simulink model "rfdc"  (R2021a)
settings: Solver=VariableStepAuto  StartTime=0.0  StopTime=10.0  RelTol=1e-3
libraries: xbsIndex_r4 x8
(part 3 of 3)

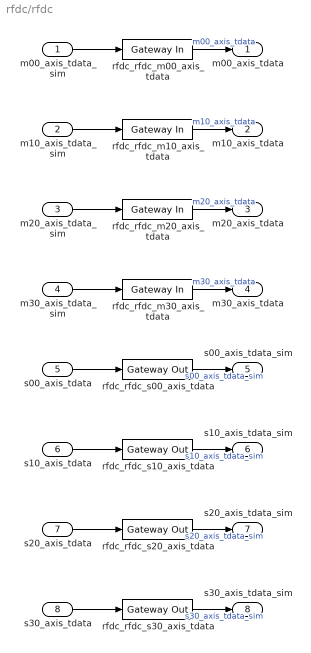
== system rfdc/rfdc ==
  m00_axis_tdata_sim : Inport
  m10_axis_tdata_sim : Inport  Port=2
  m20_axis_tdata_sim : Inport  Port=3
  m30_axis_tdata_sim : Inport  Port=4
  s00_axis_tdata : Inport  Port=5
  s10_axis_tdata : Inport  Port=6
  s20_axis_tdata : Inport  Port=7
  s30_axis_tdata : Inport  Port=8
  rfdc_rfdc_m00_axis_tdata : xbsIndex_r4/Gateway In  gui_display_data_type=Fixed-point  arith_type="Signed  (2's comp)"  n_bits=128  bin_pt=0  preci_type=Single  exp_width=8  frac_width=24  rows=1  columns=1  quantization="Round  (unbiased: +/- Inf)"  overflow=Saturate  period=1  UseAsADC=off  ADCChannel='1'  interface=None  automatic_assignment=on  address_offset=hex2dec('00')  intf_name=''  intf_description=''  default_value=0  timing_constraint=None  locs_specified=off  LOCs={}  io_standard={}  inherit_from_input=off  hdl_port=on  dbl_ovrd=off  block_type=gatewayin
  rfdc_rfdc_m10_axis_tdata : xbsIndex_r4/Gateway In  gui_display_data_type=Fixed-point  arith_type="Signed  (2's comp)"  n_bits=128  bin_pt=0  preci_type=Single  exp_width=8  frac_width=24  rows=1  columns=1  quantization="Round  (unbiased: +/- Inf)"  overflow=Saturate  period=1  UseAsADC=off  ADCChannel='1'  interface=None  automatic_assignment=on  address_offset=hex2dec('00')  intf_name=''  intf_description=''  default_value=0  timing_constraint=None  locs_specified=off  LOCs={}  io_standard={}  inherit_from_input=off  hdl_port=on  dbl_ovrd=off  block_type=gatewayin
  rfdc_rfdc_m20_axis_tdata : xbsIndex_r4/Gateway In  gui_display_data_type=Fixed-point  arith_type="Signed  (2's comp)"  n_bits=128  bin_pt=0  preci_type=Single  exp_width=8  frac_width=24  rows=1  columns=1  quantization="Round  (unbiased: +/- Inf)"  overflow=Saturate  period=1  UseAsADC=off  ADCChannel='1'  interface=None  automatic_assignment=on  address_offset=hex2dec('00')  intf_name=''  intf_description=''  default_value=0  timing_constraint=None  locs_specified=off  LOCs={}  io_standard={}  inherit_from_input=off  hdl_port=on  dbl_ovrd=off  block_type=gatewayin
  rfdc_rfdc_m30_axis_tdata : xbsIndex_r4/Gateway In  gui_display_data_type=Fixed-point  arith_type="Signed  (2's comp)"  n_bits=128  bin_pt=0  preci_type=Single  exp_width=8  frac_width=24  rows=1  columns=1  quantization="Round  (unbiased: +/- Inf)"  overflow=Saturate  period=1  UseAsADC=off  ADCChannel='1'  interface=None  automatic_assignment=on  address_offset=hex2dec('00')  intf_name=''  intf_description=''  default_value=0  timing_constraint=None  locs_specified=off  LOCs={}  io_standard={}  inherit_from_input=off  hdl_port=on  dbl_ovrd=off  block_type=gatewayin
  rfdc_rfdc_s00_axis_tdata : xbsIndex_r4/Gateway Out  inherit_from_input=off  hdl_port=on  rows=1  columns=1  UseAsDAC=off  DACChannel='1'  interface=None  automatic_assignment=on  address_offset=hex2dec('00')  intf_name=''  intf_description=''  timing_constraint=None  locs_specified=off  LOCs={}  io_standard={}  block_type=gatewayout
  rfdc_rfdc_s10_axis_tdata : xbsIndex_r4/Gateway Out  inherit_from_input=off  hdl_port=on  rows=1  columns=1  UseAsDAC=off  DACChannel='1'  interface=None  automatic_assignment=on  address_offset=hex2dec('00')  intf_name=''  intf_description=''  timing_constraint=None  locs_specified=off  LOCs={}  io_standard={}  block_type=gatewayout
  rfdc_rfdc_s20_axis_tdata : xbsIndex_r4/Gateway Out  inherit_from_input=off  hdl_port=on  rows=1  columns=1  UseAsDAC=off  DACChannel='1'  interface=None  automatic_assignment=on  address_offset=hex2dec('00')  intf_name=''  intf_description=''  timing_constraint=None  locs_specified=off  LOCs={}  io_standard={}  block_type=gatewayout
  rfdc_rfdc_s30_axis_tdata : xbsIndex_r4/Gateway Out  inherit_from_input=off  hdl_port=on  rows=1  columns=1  UseAsDAC=off  DACChannel='1'  interface=None  automatic_assignment=on  address_offset=hex2dec('00')  intf_name=''  intf_description=''  timing_constraint=None  locs_specified=off  LOCs={}  io_standard={}  block_type=gatewayout
  m00_axis_tdata : Outport
  m10_axis_tdata : Outport  Port=2
  m20_axis_tdata : Outport  Port=3
  m30_axis_tdata : Outport  Port=4
  s00_axis_tdata_sim : Outport  Port=5
  s10_axis_tdata_sim : Outport  Port=6
  s20_axis_tdata_sim : Outport  Port=7
  s30_axis_tdata_sim : Outport  Port=8
  wires:
  m00_axis_tdata_sim/1 -> rfdc_rfdc_m00_axis_tdata/1
  rfdc_rfdc_m00_axis_tdata/1 -> m00_axis_tdata/1  "m00_axis_tdata"
  m10_axis_tdata_sim/1 -> rfdc_rfdc_m10_axis_tdata/1
  rfdc_rfdc_m10_axis_tdata/1 -> m10_axis_tdata/1  "m10_axis_tdata"
  m20_axis_tdata_sim/1 -> rfdc_rfdc_m20_axis_tdata/1
  rfdc_rfdc_m20_axis_tdata/1 -> m20_axis_tdata/1  "m20_axis_tdata"
  m30_axis_tdata_sim/1 -> rfdc_rfdc_m30_axis_tdata/1
  rfdc_rfdc_m30_axis_tdata/1 -> m30_axis_tdata/1  "m30_axis_tdata"
  s00_axis_tdata/1 -> rfdc_rfdc_s00_axis_tdata/1
  rfdc_rfdc_s00_axis_tdata/1 -> s00_axis_tdata_sim/1  "s00_axis_tdata_sim"
  s10_axis_tdata/1 -> rfdc_rfdc_s10_axis_tdata/1
  rfdc_rfdc_s10_axis_tdata/1 -> s10_axis_tdata_sim/1  "s10_axis_tdata_sim"
  s20_axis_tdata/1 -> rfdc_rfdc_s20_axis_tdata/1
  rfdc_rfdc_s20_axis_tdata/1 -> s20_axis_tdata_sim/1  "s20_axis_tdata_sim"
  s30_axis_tdata/1 -> rfdc_rfdc_s30_axis_tdata/1
  rfdc_rfdc_s30_axis_tdata/1 -> s30_axis_tdata_sim/1  "s30_axis_tdata_sim"
